simulink model "EV6_LUT_FourWheel_EV6Battery77p4kWh_PowerCorrected"  (R2024a)
settings: Solver=ode4  StartTime=0  StopTime=60  FixedStep=0.001  RelTol=1e-3
PreLoadFcn:
  | VSS_BICYCLE=Simulink.Variant('Dual=0');
  | VSS_DUAL=Simulink.Variant('Dual=1');
  | Dual=1;
  | load('DriveCycle2.mat')
PostLoadFcn:
  | if any(exist('dsrtsu_mdlpostloadfcn', 'file') ~= 0), dsrtsu_mdlpostloadfcn('Execute', bdroot); end
InitFcn:
  | , if any(exist('rtifpga_mdlclblib', 'file') ~= 0), rtifpga_mdlclblib('Init', bdroot); end,
  | , if any(exist('dsmpb_private', 'file') ~= 0), dsmpb_private('dsmpb_mdlclblib', 'Init', bdroot); end,
  | load('DriveCycle2.mat')
model workspace (MAT data in the model file):
  DiffRatio = 10.65
  EV6_2023_BattBranchCapacity_Ah = 55.5236728838
  EV6_2023_BattEnergy_kWh = 77.4
  EV6_2023_BattNominalVoltage_V = 697
  EV6_2023_BattNumCellsParallel = 2
  EV6_2023_BattNumCellsSeries = 192
  EV6_2023_BattOpenVoltCapBpts = [0 0.1 0.2 0.3 0.4 0.5 0.6 0.7 0.8 0.9 1]
  EV6_2023_BattOpenVoltTbl = [2.96762142548 3.40364281191 3.47417488548 3.54470541822 3.61523441014 3.68576186124 3.75628777151 3.82681214095 3.94527005036 4.07101207308 4.2120755254]
  EV6_2023_BattPackCapacity_Ah = 111.047345768
  EV6_2023_BattResistSocBpts = [0 0.2 0.4 0.6 0.8 1]
  EV6_2023_BattResistTbl = [0.0163620057716 0.0118174152018 0.00807187352333 0.00375663957972 0.00266904525531 0.00103635901355 0.0019014404175 0.0172368903217 0.0121226074867 0.00758541551769 0.00474065349228 0.00337561163613 ... (42 elements, 7x6)]
  EV6_2023_BattResistTempBpts = [243.1 253.1 263.1 273.1 283.1 298.1 313.1]
  EV6_2023_InitialPackOCV_V = 726.471714233
  EV6_2023_InitialSOC = 0.638878863672
  EV6_BattCellCapacity_Ah = 60.3
  EV6_BattInitialSOC = 0.638878863672
  EV6_BattOCV_Cell_V = [2.96762142548 3.40364281191 3.47417488548 3.54470541822 3.61523441014 3.68576186124 3.75628777151 3.82681214095 3.94527005036 4.07101207308 4.2120755254]
  EV6_BattOCV_SOC = [0 0.1 0.2 0.3 0.4 0.5 0.6 0.7 0.8 0.9 1]
  EV6_BattPackCapacity_Ah = 120.6
  EV6_BattParallelCells = 2
  EV6_BattResistanceSOC = [0 0.2 0.4 0.6 0.8 1]
  EV6_BattResistanceTable_Ohm = [0.0163620057716 0.0118174152018 0.00807187352333 0.00375663957972 0.00266904525531 0.00103635901355 0.0019014404175 0.0172368903217 0.0121226074867 0.00758541551769 0.00474065349228 0.00337561163613 ... (42 elements, 7x6)]
  EV6_BattResistanceTemp_K = [243.1 253.1 263.1 273.1 283.1 298.1 313.1]
  EV6_BattSeriesCells = 192
  EV6_FinalDriveRatio = 10.65
  EV6_TargetPackResistance_Ohm = 0.132763804608
  Gas = 0.383333333333
undefined symbols (not defined in the file): accel_bp_mps2, AccelCmd, ActTqLF_Nm_, ActTqLR_Nm_, ActTqRF_Nm_, ActTqRR_Nm_, BattChargeLimitMaxPwr, BattChargeLimitSocBpts, BattChargeLimitTbl, BattDischargeLimitSocBpts, BattDischargeLimitTbl, BattDischargeMaxPwr, BrakeMaxPrs, BrakeMaxTrq, ChassisDistCg2FrontAxle, ChassisDistCg2RearAxle, ChassisVehMass, CltchCmd, CoastDown, DecelCmd, DiscIntNeverNeededParam, EnvGravCnst, EnvPrs, EnvTemp, EV6_RegenTorqueGain, EV6_TractionTorqueGain, front_share_regen_3d, front_share_traction_3d, FuelSpecificGrav, GearCmd, h, InitStates, lgSw, limitedMCT, MCT, MtrEffSpdBpts, MtrEffTbl, MtrEffTrqBpts, MtrPwrMax, MtrTrqMax, out_1, pMCT, RealSimPara, Ref_speed, Ref_time, regen_torque_bp_Nm, speed_bp_kph, SteeringCmd, SupvsryCtrlRegenBrkCutOffTbl, SupvsryCtrlRegenSpdBpts, TestScnrioCycleNum, traction_torque_bp_Nm, US06, VEH
libraries: VSIGenLib x65, simulink x54, etargetslib x38, dsmpblib x24, vehdynlibtire x12, autolibshared x11, vehdynlibsuspension x7, vehdynlibtirecommon x7, autolibpowerinfoutils x6, autolibutils x5, autolibsharedcoupling x4, autolibmappedmotor x4
(part 10 of 19)

== system EV6_LUT_FourWheel_EV6Battery77p4kWh_PowerCorrected/Vehicle Under Test1/Vehicle/Powertrain Supervisory Controller /Engine Torque Command/Motor Torque Arbitration and Power Management/Power Management ==
  note: Power Management algorithm:
      | - Estimate Elec power based on mech power using efficiency map
      | - Check if Elec power is within battery power limits
      | - If power within limit , use motor torque command
      | - If power limit exceeded, use limited motor torque
      | - For low Mot Spd, MotPwrReq will be a small number.  Pass through torque command until Mot Spd > 2.
  BattPwrDischrgLmt : Inport
  BattPwrChrgLmt : Inport  Port=2
  MotSpd : Inport  Port=3
  MotTrqCmd : Inport  Port=4
  Abs : Abs  SaturateOnIntegerOverflow=off
  Check Within Limits : Subsystem
  Compare To Constant : simulink/Logic and Bit Operations/Compare To Constant  relop=<  const=2  OutDataTypeStr=boolean
  ElecToMechPwr : Product  Inputs=*/
  Mech to Elec Power Estimate : Subsystem
  MechPwrToTrq : Product  Inputs=*/
  Switch : Switch  Criteria=u2 > Threshold  SaturateOnIntegerOverflow=off  InputSameDT=off
  Switch1 : Switch  Criteria=u2 > Threshold  SaturateOnIntegerOverflow=off  InputSameDT=off
  Torque Limit : Subsystem
  div0protect - poly : autolibutils/div0protect - poly  thresh=2  ZeroCross1=on  aMode=aMode
  MotTrqCmdFinal : Outport  VectorParamsAs1DForOutWhenUnconnected=off
  wires:
  MotSpd/1 -> Torque Limit/2(MotSpd), div0protect - poly/1, Mech to Elec Power Estimate/2(MotSpd), Abs/1
  MotTrqCmd/1 -> Switch/1, Switch1/1, Mech to Elec Power Estimate/1(MotTrqCmd)
  div0protect - poly/1 -> MechPwrToTrq/2
  Mech to Elec Power Estimate/2(Eff2k) -> ElecToMechPwr/2
  ElecToMechPwr/1 -> MechPwrToTrq/1
  MechPwrToTrq/1 -> Switch/3
  Torque Limit/1(MotTrqCmd) -> MotTrqCmdFinal/1
  BattPwrDischrgLmt/1 -> Check Within Limits/1(up)
  Mech to Elec Power Estimate/1(MotPwrElecReq) -> Check Within Limits/2(u)
  BattPwrChrgLmt/1 -> Check Within Limits/3(lo)
  Check Within Limits/2(y) -> ElecToMechPwr/1
  Switch/1 -> Switch1/3
  Check Within Limits/1(InLimit) -> Switch/2
  Switch1/1 -> Torque Limit/1(MotTrq)
  Abs/1 -> Compare To Constant/1
  Compare To Constant/1 -> Switch1/2

== system EV6_LUT_FourWheel_EV6Battery77p4kWh_PowerCorrected/Vehicle Under Test1/Vehicle/Rototest and ORNL Interface/From Rototest/RotoTestEthRX/Depacker ==
  SysStsBits : Inport
  Extract Bits1 : simulink/Logic and Bit Operations/Extract Bits  bitsToExtract=Range of bits  numBits=8  bitIdxRange=[7]  outScalingMode=Preserve fixed-point scaling
  Extract Bits10 : simulink/Logic and Bit Operations/Extract Bits  bitsToExtract=Range of bits  numBits=8  bitIdxRange=[9]  outScalingMode=Preserve fixed-point scaling
  Extract Bits11 : simulink/Logic and Bit Operations/Extract Bits  bitsToExtract=Range of bits  numBits=8  bitIdxRange=[10]  outScalingMode=Preserve fixed-point scaling
  Extract Bits12 : simulink/Logic and Bit Operations/Extract Bits  bitsToExtract=Range of bits  numBits=8  bitIdxRange=[11]  outScalingMode=Preserve fixed-point scaling
  Extract Bits13 : simulink/Logic and Bit Operations/Extract Bits  bitsToExtract=Range of bits  numBits=8  bitIdxRange=[12]  outScalingMode=Preserve fixed-point scaling
  Extract Bits14 : simulink/Logic and Bit Operations/Extract Bits  bitsToExtract=Range of bits  numBits=8  bitIdxRange=[13]  outScalingMode=Preserve fixed-point scaling
  Extract Bits15 : simulink/Logic and Bit Operations/Extract Bits  bitsToExtract=Range of bits  numBits=8  bitIdxRange=[14]  outScalingMode=Preserve fixed-point scaling
  Extract Bits16 : simulink/Logic and Bit Operations/Extract Bits  bitsToExtract=Range of bits  numBits=8  bitIdxRange=[15]  outScalingMode=Preserve fixed-point scaling
  Extract Bits2 : simulink/Logic and Bit Operations/Extract Bits  bitsToExtract=Range of bits  numBits=8  bitIdxRange=[6]  outScalingMode=Preserve fixed-point scaling
  Extract Bits3 : simulink/Logic and Bit Operations/Extract Bits  bitsToExtract=Range of bits  numBits=8  bitIdxRange=[5]  outScalingMode=Preserve fixed-point scaling
  Extract Bits4 : simulink/Logic and Bit Operations/Extract Bits  bitsToExtract=Range of bits  numBits=8  bitIdxRange=[4]  outScalingMode=Preserve fixed-point scaling
  Extract Bits5 : simulink/Logic and Bit Operations/Extract Bits  bitsToExtract=Range of bits  numBits=8  bitIdxRange=[3]  outScalingMode=Preserve fixed-point scaling
  Extract Bits6 : simulink/Logic and Bit Operations/Extract Bits  bitsToExtract=Range of bits  numBits=8  bitIdxRange=[2]  outScalingMode=Preserve fixed-point scaling
  Extract Bits7 : simulink/Logic and Bit Operations/Extract Bits  bitsToExtract=Range of bits  numBits=8  bitIdxRange=[1]  outScalingMode=Preserve fixed-point scaling
  Extract Bits8 : simulink/Logic and Bit Operations/Extract Bits  bitsToExtract=Range of bits  numBits=8  bitIdxRange=[0]  outScalingMode=Preserve fixed-point scaling
  Extract Bits9 : simulink/Logic and Bit Operations/Extract Bits  bitsToExtract=Range of bits  numBits=8  bitIdxRange=[8]  outScalingMode=Preserve fixed-point scaling
  Gain : Gain  Gain=1/128
  Gain1 : Gain  Gain=1/64
  Gain10 : Gain  Gain=1/1024
  Gain11 : Gain  Gain=1/2048
  Gain12 : Gain  Gain=1/4096
  Gain13 : Gain  Gain=1/8192
  Gain14 : Gain  Gain=1/16384
  Gain15 : Gain  Gain=1/32768
  Gain2 : Gain  Gain=1/32
  Gain3 : Gain  Gain=1/16
  Gain4 : Gain  Gain=1/8
  Gain5 : Gain  Gain=1/4
  Gain6 : Gain  Gain=1/2
  Gain7 : Gain  Gain=1/1
  Gain8 : Gain  Gain=1/256
  Gain9 : Gain  Gain=1/512
  Header : VSIGenLib/Header  not=''
  Terminator{,1..8} (9 alike) : Terminator
  FaultActive : Outport
  WarningsActive : Outport  Port=2
  SpTqRR : Outport  Port=3
  SpTqLR : Outport  Port=4
  SpTqRF : Outport  Port=5
  SpTqLF : Outport  Port=6
  SystemActive : Outport  Port=7
  wires:
  Extract Bits6/1 -> Gain5/1
  Extract Bits4/1 -> Gain3/1
  Extract Bits8/1 -> Gain7/1
  Extract Bits7/1 -> Gain6/1
  Extract Bits3/1 -> Gain2/1
  Extract Bits1/1 -> Gain/1
  Extract Bits5/1 -> Gain4/1
  Extract Bits2/1 -> Gain1/1
  Extract Bits10/1 -> Gain9/1
  Extract Bits9/1 -> Gain8/1
  Extract Bits11/1 -> Gain10/1
  Extract Bits12/1 -> Gain11/1
  Extract Bits13/1 -> Gain12/1
  Extract Bits15/1 -> Gain14/1
  Extract Bits14/1 -> Gain13/1
  Extract Bits16/1 -> Gain15/1
  SysStsBits/1 -> Extract Bits1/1, Extract Bits2/1, Extract Bits3/1, Extract Bits4/1, Extract Bits5/1, Extract Bits6/1, Extract Bits7/1, Extract Bits8/1, Extract Bits11/1, Extract Bits12/1, Extract Bits13/1, Extract Bits14/1, Extract Bits15/1, Extract Bits16/1, Extract Bits10/1, Extract Bits9/1
  Gain15/1 -> Terminator6/1  "Reserved"
  Gain13/1 -> Terminator8/1  "Reserved"
  Gain14/1 -> Terminator7/1  "Reserved"
  Gain12/1 -> SpTqRR/1  "SpTqRR"
  Gain11/1 -> SpTqLR/1  "SpTqLR"
  Gain10/1 -> SpTqRF/1  "SpTqRF"
  Gain9/1 -> SpTqLF/1  "SpTqLF"
  Gain8/1 -> SystemActive/1  "SystemActive"
  Gain7/1 -> Terminator5/1  "Reserved"
  Gain/1 -> FaultActive/1  "FaultActive"
  Gain1/1 -> WarningsActive/1  "WarningsActive"
  Gain2/1 -> Terminator/1  "Reserved"
  Gain4/1 -> Terminator2/1  "Reserved"
  Gain3/1 -> Terminator1/1  "Reserved"
  Gain6/1 -> Terminator4/1  "Reserved"
  Gain5/1 -> Terminator3/1  "Reserved"

== system EV6_LUT_FourWheel_EV6Battery77p4kWh_PowerCorrected/Vehicle Under Test1/Vehicle/Rototest and ORNL Interface/Get Wheel Spd Cmd Based on Wheel Dynamics/Whl Dynamics & Format CM Powertrain Signal/Diff Trq ==
  In1 : Inport
  Constant : Constant  Value=4.1
  Gain10 : Gain  Gain=0.5
  Product : Product  RndMeth=Zero
  Out1 : Outport
  wires:
  Product/1 -> Gain10/1  "DiffTrq"
  In1/1 -> Product/2
  Constant/1 -> Product/1
  Gain10/1 -> Out1/1

== system EV6_LUT_FourWheel_EV6Battery77p4kWh_PowerCorrected/Vehicle Under Test1/Vehicle/Rototest and ORNL Interface/Get Wheel Spd Cmd Based on Wheel Dynamics/Whl Dynamics & Format CM Powertrain Signal/Subsystem ==
  BrakeTorq : Inport
  <Car Trq_T2WFL> : Inport  Port=2
  AxlTorq : Inport  Port=3
  Fx : Inport  Port=4
  Add1 : Sum  Inputs=--+
  Add2 : Sum  Inputs=-+
  Constant : Constant  Value=0
  Constant9 : Constant  Value=0.3135
  MATLAB Function : MATLAB Function  TreatAsAtomicUnit=on
  Memory : Memory
  Output Damping : Gain  Gain=0  SaturateOnIntegerOverflow=on  OutDataTypeStr=Inherit: Same as input  ParamDataTypeStr=Inherit: Same as input
  Product3 : Product  Inputs=**
  Saturation : Saturate  UpperLimit=inf  LowerLimit=0  ZeroCross=off
  Sum : Sum  Inputs=--
  Sum3 : Sum  Inputs=-++
  Switch : Switch  Criteria=u2 > Threshold  SaturateOnIntegerOverflow=off  InputSameDT=off
  WheelInertia : Subsystem
  WheelInertia1 : Subsystem
  omega wheel : Integrator  ContinuousStateAttributes='omegaWheel'
  rotv FL : Outport
  wires:
  [Fx1] -> Product3/1
  Sum/1 -> Switch/3
  WheelInertia1/1(axleTorq) -> Sum/1  "rota"
  Output Damping/1 -> Sum/2
  omega wheel/1 -> rotv FL/1, Output Damping/1, Memory/1
  Switch/1 -> omega wheel/1
  Add1/1 -> WheelInertia1/1(In1)
  Saturation/1 -> Product3/2
  Product3/1 -> Add1/3
  <Car Trq_T2WFL>/1 -> Sum3/2, Add1/2
  AxlTorq/1 -> Sum3/3, MATLAB Function/1(axleTorq), Add1/1
  Constant9/1 -> Add2/2
  [RhoZ1] -> Add2/1
  Add2/1 -> Saturation/1
  Memory/1 -> MATLAB Function/2(wheelSpd)
  Constant/1 -> Switch/1
  MATLAB Function/1(switchFlag) -> Switch/2  "Flag1"
  BrakeTorq/1 -> Sum3/1
  Sum3/1 -> WheelInertia/1(In1)

== system EV6_LUT_FourWheel_EV6Battery77p4kWh_PowerCorrected/Vehicle Under Test1/Vehicle/Rototest and ORNL Interface/Get Wheel Spd Cmd Based on Wheel Dynamics/Whl Dynamics & Format CM Powertrain Signal/Subsystem1 ==
  BrakeTorq : Inport
  <Car Trq_T2WFL> : Inport  Port=2
  AxlTorq : Inport  Port=3
  Discrete-Time Integrator : DiscreteIntegrator  IntegratorMethod=Integration: Backward Euler  InitialCondition=0/3.6/0.3235  SampleTime=0.001  ICPrevOutput=DiscIntNeverNeededParam  ICPrevScaledInput=DiscIntNeverNeededParam
  Sum3 : Sum  Inputs=-++
  WheelInertia : Subsystem
  rotv FL : Outport
  wires:
  WheelInertia/1(Out1) -> Discrete-Time Integrator/1
  Discrete-Time Integrator/1 -> rotv FL/1  "rotv FL"
  BrakeTorq/1 -> Sum3/1
  <Car Trq_T2WFL>/1 -> Sum3/2
  AxlTorq/1 -> Sum3/3
  Sum3/1 -> WheelInertia/1(In1)

== system EV6_LUT_FourWheel_EV6Battery77p4kWh_PowerCorrected/Vehicle Under Test1/Vehicle/Rototest and ORNL Interface/Get Wheel Spd Cmd Based on Wheel Dynamics/Whl Dynamics & Format CM Powertrain Signal/Subsystem2 ==
  BrakeTorq : Inport
  <Car Trq_T2WFR> : Inport  Port=2
  AxlTorq : Inport  Port=3
  Fx : Inport  Port=4
  Add1 : Sum  Inputs=--+
  Add2 : Sum  Inputs=-+
  Constant : Constant  Value=0
  Constant9 : Constant  Value=0.3135
  MATLAB Function : MATLAB Function  TreatAsAtomicUnit=on
  Memory : Memory
  Output Damping : Gain  Gain=-1  SaturateOnIntegerOverflow=on  OutDataTypeStr=Inherit: Same as input  ParamDataTypeStr=Inherit: Same as input
  Product3 : Product  Inputs=**
  Saturation : Saturate  UpperLimit=inf  LowerLimit=0  ZeroCross=off
  Sum3 : Sum  Inputs=-++
  Switch : Switch  Criteria=u2 > Threshold  SaturateOnIntegerOverflow=off  InputSameDT=off
  WheelInertia : Subsystem
  WheelInertia1 : Subsystem
  omega wheel : Integrator  ContinuousStateAttributes='omegaWheel'
  rotv FR : Outport
  wires:
  [Fx2] -> Product3/1
  Output Damping/1 -> Switch/3
  Switch/1 -> omega wheel/1
  omega wheel/1 -> rotv FR/1, Memory/1
  AxlTorq/1 -> Sum3/3, MATLAB Function/1(axleTorq), Add1/1
  Add2/1 -> Saturation/1
  Saturation/1 -> Product3/2
  [RhoZ2] -> Add2/1
  Add1/1 -> WheelInertia1/1(In1)
  Constant9/1 -> Add2/2
  <Car Trq_T2WFR>/1 -> Sum3/2, Add1/2
  Product3/1 -> Add1/3
  WheelInertia1/1(Out1) -> Output Damping/1  "rota"
  Memory/1 -> MATLAB Function/2(wheelSpd)
  Sum3/1 -> WheelInertia/1(In1)
  BrakeTorq/1 -> Sum3/1
  Constant/1 -> Switch/1
  MATLAB Function/1(switchFlag) -> Switch/2

== system EV6_LUT_FourWheel_EV6Battery77p4kWh_PowerCorrected/Vehicle Under Test1/Vehicle/Rototest and ORNL Interface/Get Wheel Spd Cmd Based on Wheel Dynamics/Whl Dynamics & Format CM Powertrain Signal/Subsystem3 ==
  BrakeTorq : Inport
  <Car Trq_T2WRL> : Inport  Port=2
  AxlTorq : Inport  Port=3
  Fx : Inport  Port=4
  FWSpd : Inport  Port=5
  Add1 : Sum  Inputs=--+
  Add2 : Sum  Inputs=-+
  Constant : Constant  Value=0
  Constant9 : Constant  Value=0.3135
  MATLAB Function : MATLAB Function  TreatAsAtomicUnit=on
  Memory : Memory
  Output Damping : Gain  Gain=0  SaturateOnIntegerOverflow=on  OutDataTypeStr=Inherit: Same as input  ParamDataTypeStr=Inherit: Same as input
  Product3 : Product  Inputs=**
  Saturation : Saturate  UpperLimit=inf  LowerLimit=0  ZeroCross=off
  Sum : Sum  Inputs=--
  Sum3 : Sum  Inputs=-++
  Switch : Switch  Criteria=u2 > Threshold  SaturateOnIntegerOverflow=off  InputSameDT=off
  WheelInertia : Subsystem
  WheelInertia1 : Subsystem
  omega wheel : Integrator  ContinuousStateAttributes='omegaWheel'
  rotv RL : Outport
  wires:
  WheelInertia1/1(axleTorq) -> Sum/1  "rota"
  omega wheel/1 -> rotv RL/1, Output Damping/1
  Output Damping/1 -> Sum/2
  [Fx3] -> Product3/1
  Switch/1 -> omega wheel/1
  Sum/1 -> Switch/3
  FWSpd/1 -> MATLAB Function/2(wheelSpd)
  AxlTorq/1 -> Sum3/3, MATLAB Function/1(axleTorq), Add1/1
  Add2/1 -> Saturation/1
  Saturation/1 -> Product3/2
  [RhoZ3] -> Add2/1
  Add1/1 -> WheelInertia1/1(In1)
  Constant9/1 -> Add2/2
  <Car Trq_T2WRL>/1 -> Add1/2, Sum3/2
  Product3/1 -> Add1/3
  Sum3/1 -> WheelInertia/1(In1)
  BrakeTorq/1 -> Sum3/1
  Constant/1 -> Switch/1
  MATLAB Function/1(switchFlag) -> Switch/2

== system EV6_LUT_FourWheel_EV6Battery77p4kWh_PowerCorrected/Vehicle Under Test1/Vehicle/Rototest and ORNL Interface/Get Wheel Spd Cmd Based on Wheel Dynamics/Whl Dynamics & Format CM Powertrain Signal/Subsystem4 ==
  BrakeTorq : Inport
  <Car Trq_T2WRR> : Inport  Port=2
  AxlTorq : Inport  Port=3
  Fx : Inport  Port=4
  FWSpd : Inport  Port=5
  Add1 : Sum  Inputs=--+
  Add2 : Sum  Inputs=-+
  Constant : Constant  Value=0
  Constant9 : Constant  Value=0.3135
  Gain : Gain  Gain=-1
  MATLAB Function : MATLAB Function  TreatAsAtomicUnit=on
  Memory : Memory
  Product3 : Product  Inputs=**
  Saturation : Saturate  UpperLimit=inf  LowerLimit=0  ZeroCross=off
  Sum3 : Sum  Inputs=-++
  Switch : Switch  Criteria=u2 > Threshold  SaturateOnIntegerOverflow=off  InputSameDT=off
  WheelInertia : Subsystem
  WheelInertia1 : Subsystem
  omega wheel : Integrator  ContinuousStateAttributes='omegaWheel'
  rotv RR : Outport
  wires:
  WheelInertia1/1(axleTorq) -> Gain/1  "rota"
  [Fx4] -> Product3/1
  omega wheel/1 -> rotv RR/1
  Switch/1 -> omega wheel/1
  Gain/1 -> Switch/3
  FWSpd/1 -> MATLAB Function/2(wheelSpd)
  AxlTorq/1 -> Sum3/3, MATLAB Function/1(axleTorq), Add1/1
  Add2/1 -> Saturation/1
  Saturation/1 -> Product3/2
  [RhoZ4] -> Add2/1
  Add1/1 -> WheelInertia1/1(In1)
  Constant9/1 -> Add2/2
  <Car Trq_T2WRR>/1 -> Sum3/2, Add1/2
  Product3/1 -> Add1/3
  Sum3/1 -> WheelInertia/1(In1)
  BrakeTorq/1 -> Sum3/1
  Constant/1 -> Switch/1
  MATLAB Function/1(switchFlag) -> Switch/2

== system EV6_LUT_FourWheel_EV6Battery77p4kWh_PowerCorrected/Vehicle Under Test1/Vehicle/Rototest and ORNL Interface/Get Wheel Spd Cmd Based on Wheel Dynamics/Whl Dynamics & Format CM Powertrain Signal/Subsystem5 ==
  In1 : Inport
  <Car Trq_T2WFR> : Inport  Port=2
  In3 : Inport  Port=3
  Discrete-Time Integrator1 : DiscreteIntegrator  IntegratorMethod=Integration: Backward Euler  InitialCondition=0/3.6/0.3235  SampleTime=0.001  ICPrevOutput=DiscIntNeverNeededParam  ICPrevScaledInput=DiscIntNeverNeededParam
  Sum2 : Sum  Inputs=-++
  WheelInertia1 : Subsystem
  rotv FR : Outport
  wires:
  Discrete-Time Integrator1/1 -> rotv FR/1  "rotv FR"
  In1/1 -> Sum2/1
  WheelInertia1/1(Out1) -> Discrete-Time Integrator1/1  "rota"
  In3/1 -> Sum2/3
  Sum2/1 -> WheelInertia1/1(In1)
  <Car Trq_T2WFR>/1 -> Sum2/2

== system EV6_LUT_FourWheel_EV6Battery77p4kWh_PowerCorrected/Vehicle Under Test1/Vehicle/Rototest and ORNL Interface/Get Wheel Spd Cmd Based on Wheel Dynamics/Whl Dynamics & Format CM Powertrain Signal/Subsystem6 ==
  In1 : Inport
  <Car Trq_T2WRL> : Inport  Port=2
  In3 : Inport  Port=3
  Discrete-Time Integrator2 : DiscreteIntegrator  IntegratorMethod=Integration: Backward Euler  InitialCondition=0/3.6/0.3235  SampleTime=0.001  ICPrevOutput=DiscIntNeverNeededParam  ICPrevScaledInput=DiscIntNeverNeededParam
  Sum : Sum  Inputs=-++
  WheelInertia2 : Subsystem
  rotv RL : Outport
  wires:
  In1/1 -> Sum/1
  Discrete-Time Integrator2/1 -> rotv RL/1  "rotv RL"
  Sum/1 -> WheelInertia2/1(In1)
  <Car Trq_T2WRL>/1 -> Sum/2
  WheelInertia2/1(Out1) -> Discrete-Time Integrator2/1  "rota"
  In3/1 -> Sum/3

== system EV6_LUT_FourWheel_EV6Battery77p4kWh_PowerCorrected/Vehicle Under Test1/Vehicle/Rototest and ORNL Interface/Get Wheel Spd Cmd Based on Wheel Dynamics/Whl Dynamics & Format CM Powertrain Signal/Subsystem7 ==
  In1 : Inport
  <Car Trq_T2WRR> : Inport  Port=2
  In3 : Inport  Port=3
  Discrete-Time Integrator3 : DiscreteIntegrator  IntegratorMethod=Integration: Backward Euler  InitialCondition=0/3.6/0.3235  SampleTime=0.001  ICPrevOutput=DiscIntNeverNeededParam  ICPrevScaledInput=DiscIntNeverNeededParam
  Sum1 : Sum  Inputs=-++
  WheelInertia3 : Subsystem
  rotv RR : Outport
  wires:
  Discrete-Time Integrator3/1 -> rotv RR/1  "rotv RR"
  In1/1 -> Sum1/1
  <Car Trq_T2WRR>/1 -> Sum1/2
  In3/1 -> Sum1/3
  WheelInertia3/1(Out1) -> Discrete-Time Integrator3/1  "rota"
  Sum1/1 -> WheelInertia3/1(In1)

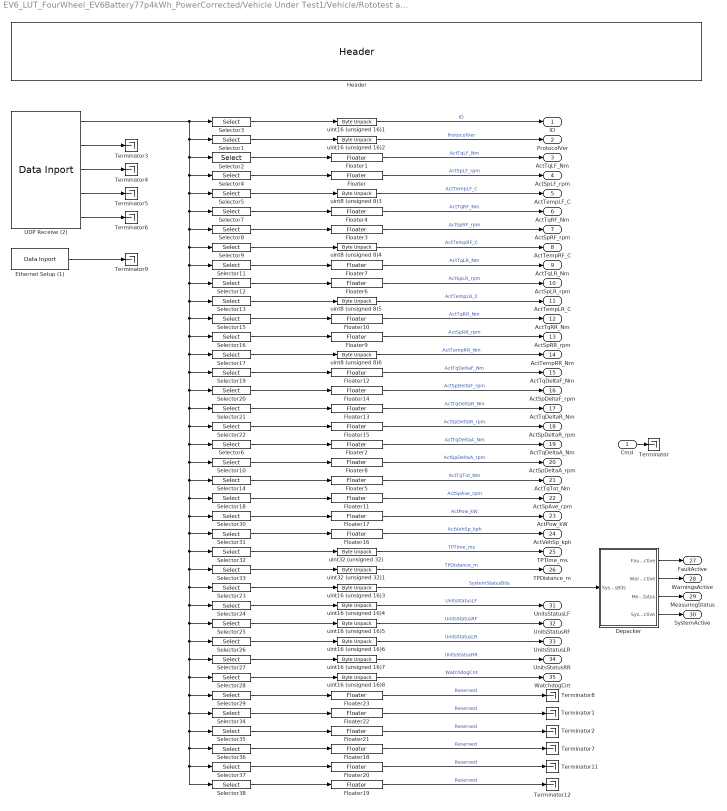
== system EV6_LUT_FourWheel_EV6Battery77p4kWh_PowerCorrected/Vehicle Under Test1/Vehicle/Rototest and ORNL Interface/To Rototest with Band-Aid/Logging/RotoTestEthRXLogging ==
  Cmd : Inport
  Depacker : Subsystem
  Ethernet Setup (1) : dsmpblib/Data Inport  Priority=10000
      settings: SourceProductName=dSPACE Model Interface Package for Simulink (MIPS)
  Floater{,1..23} (24 alike) : VSIGenLib/Floater  SystemSampleTime=-1  VariantActivationTime=update diagram  AllowFlexibleInterface=on  Latency=0  AutoFrameSizeCalculation=off
  Header : VSIGenLib/Header  not=''
  Selector1 : Selector  IndexMode=Zero-based  InputPortWidth=124  IndexOptions=Index vector (dialog)  Indices=[3 2]  OutputSizes=1
  Selector10 : Selector  IndexMode=Zero-based  InputPortWidth=124  IndexOptions=Index vector (dialog)  Indices=[63 62 61 60]  OutputSizes=1
  Selector11 : Selector  IndexMode=Zero-based  InputPortWidth=124  IndexOptions=Index vector (dialog)  Indices=[25 24 23 22]  OutputSizes=1
  Selector12 : Selector  IndexMode=Zero-based  InputPortWidth=124  IndexOptions=Index vector (dialog)  Indices=[29 28 27 26]  OutputSizes=1
  Selector13 : Selector  IndexMode=Zero-based  InputPortWidth=124  IndexOptions=Index vector (dialog)  Indices=[30]  OutputSizes=1
  Selector14 : Selector  IndexMode=Zero-based  InputPortWidth=124  IndexOptions=Index vector (dialog)  Indices=[67 66 65 64]  OutputSizes=1
  Selector15 : Selector  IndexMode=Zero-based  InputPortWidth=124  IndexOptions=Index vector (dialog)  Indices=[34 33 32 31]  OutputSizes=1
  Selector16 : Selector  IndexMode=Zero-based  InputPortWidth=124  IndexOptions=Index vector (dialog)  Indices=[38 37 36 35]  OutputSizes=1
  Selector17 : Selector  IndexMode=Zero-based  InputPortWidth=124  IndexOptions=Index vector (dialog)  Indices=[39]  OutputSizes=1
  Selector18 : Selector  IndexMode=Zero-based  InputPortWidth=124  IndexOptions=Index vector (dialog)  Indices=[71 70 69 68]  OutputSizes=1
  Selector19 : Selector  IndexMode=Zero-based  InputPortWidth=124  IndexOptions=Index vector (dialog)  Indices=[43 42 41 40]  OutputSizes=1
  Selector2 : Selector  IndexMode=Zero-based  InputPortWidth=124  IndexOptions=Index vector (dialog)  Indices=[7 6 5 4]  OutputSizes=1
  Selector20 : Selector  IndexMode=Zero-based  InputPortWidth=124  IndexOptions=Index vector (dialog)  Indices=[47 46 45 44]  OutputSizes=1
  Selector21 : Selector  IndexMode=Zero-based  InputPortWidth=124  IndexOptions=Index vector (dialog)  Indices=[51 50 49 48]  OutputSizes=1
  Selector22 : Selector  IndexMode=Zero-based  InputPortWidth=124  IndexOptions=Index vector (dialog)  Indices=[55 54 53 52]  OutputSizes=1
  Selector23 : Selector  IndexMode=Zero-based  InputPortWidth=124  IndexOptions=Index vector (dialog)  Indices=[89 88]  OutputSizes=1
  Selector24 : Selector  IndexMode=Zero-based  InputPortWidth=124  IndexOptions=Index vector (dialog)  Indices=[91 90]  OutputSizes=1
  Selector25 : Selector  IndexMode=Zero-based  InputPortWidth=124  IndexOptions=Index vector (dialog)  Indices=[93 92]  OutputSizes=1
  Selector26 : Selector  IndexMode=Zero-based  InputPortWidth=124  IndexOptions=Index vector (dialog)  Indices=[95 94]  OutputSizes=1
  Selector27 : Selector  IndexMode=Zero-based  InputPortWidth=124  IndexOptions=Index vector (dialog)  Indices=[97 96]  OutputSizes=1
  Selector28 : Selector  IndexMode=Zero-based  InputPortWidth=124  IndexOptions=Index vector (dialog)  Indices=[99 98]  OutputSizes=1
  Selector29 : Selector  IndexMode=Zero-based  InputPortWidth=124  IndexOptions=Index vector (dialog)  Indices=[103 102 101 100]  OutputSizes=1
  Selector3 : Selector  IndexMode=Zero-based  InputPortWidth=124  IndexOptions=Index vector (dialog)  Indices=[1 0]  OutputSizes=1
  Selector30 : Selector  IndexMode=Zero-based  InputPortWidth=124  IndexOptions=Index vector (dialog)  Indices=[67 66 65 64]  OutputSizes=1
  Selector31 : Selector  IndexMode=Zero-based  InputPortWidth=124  IndexOptions=Index vector (dialog)  Indices=[71 70 69 68]  OutputSizes=1
  Selector32 : Selector  IndexMode=Zero-based  InputPortWidth=124  IndexOptions=Index vector (dialog)  Indices=[83 82 81 80]  OutputSizes=1
  Selector33 : Selector  IndexMode=Zero-based  InputPortWidth=124  IndexOptions=Index vector (dialog)  Indices=[87 86 85 84]  OutputSizes=1
  Selector34 : Selector  IndexMode=Zero-based  InputPortWidth=124  IndexOptions=Index vector (dialog)  Indices=[107 106 105 104]  OutputSizes=1
  Selector35 : Selector  IndexMode=Zero-based  InputPortWidth=124  IndexOptions=Index vector (dialog)  Indices=[111 110 109 108]  OutputSizes=1
  Selector36 : Selector  IndexMode=Zero-based  InputPortWidth=124  IndexOptions=Index vector (dialog)  Indices=[115 114 113 112]  OutputSizes=1
  Selector37 : Selector  IndexMode=Zero-based  InputPortWidth=124  IndexOptions=Index vector (dialog)  Indices=[119 118 117 116]  OutputSizes=1
  Selector38 : Selector  IndexMode=Zero-based  InputPortWidth=124  IndexOptions=Index vector (dialog)  Indices=[123 122 121 120]  OutputSizes=1
  Selector4 : Selector  IndexMode=Zero-based  InputPortWidth=124  IndexOptions=Index vector (dialog)  Indices=[11 10 9 8]  OutputSizes=1
  Selector5 : Selector  IndexMode=Zero-based  InputPortWidth=124  IndexOptions=Index vector (dialog)  Indices=[12]  OutputSizes=1
  Selector6 : Selector  IndexMode=Zero-based  InputPortWidth=124  IndexOptions=Index vector (dialog)  Indices=[59 58 57 56]  OutputSizes=1
  Selector7 : Selector  IndexMode=Zero-based  InputPortWidth=124  IndexOptions=Index vector (dialog)  Indices=[16 15 14 13]  OutputSizes=1
  Selector8 : Selector  IndexMode=Zero-based  InputPortWidth=124  IndexOptions=Index vector (dialog)  Indices=[20 19 18 17]  OutputSizes=1
  Selector9 : Selector  IndexMode=Zero-based  InputPortWidth=124  IndexOptions=Index vector (dialog)  Indices=[21]  OutputSizes=1
  Terminator{,1..9,11..12} (12 alike) : Terminator
  UDP Receive (2) : dsmpblib/Data Inport  Priority=10000
      settings: SourceProductName=dSPACE Model Interface Package for Simulink (MIPS)
  uint16 (unsigned 16){1..8} (8 alike) : etargetslib/Byte Unpack  dimensions={[1]}  datatypes={'uint16'}  byteAlign=1
  uint32 (unsigned 32) : etargetslib/Byte Unpack  dimensions={[1]}  datatypes={'uint32'}  byteAlign=1
  uint32 (unsigned 32)1 : etargetslib/Byte Unpack  dimensions={[1]}  datatypes={'uint32'}  byteAlign=1
  uint8 (unsigned 8){3..6} (4 alike) : etargetslib/Byte Unpack  dimensions={[1]}  datatypes={'uint8'}  byteAlign=1
  ID : Outport
  ProtocolVer : Outport  Port=2
  ActTqLF_Nm : Outport  Port=3
  ActSpLF_rpm : Outport  Port=4
  ActTempLF_C : Outport  Port=5
  ActTqRF_Nm : Outport  Port=6
  ActSpRF_rpm : Outport  Port=7
  ActTempRF_C : Outport  Port=8
  ActTqLR_Nm : Outport  Port=9
  ActSpLR_rpm : Outport  Port=10
  ActTempLR_C : Outport  Port=11
  ActTqRR_Nm : Outport  Port=12
  ActSpRR_rpm : Outport  Port=13
  ActTempRR_Nm : Outport  Port=14
  ActTqDeltaF_Nm : Outport  Port=15
  ActSpDeltaF_rpm : Outport  Port=16
  ActTqDeltaR_Nm : Outport  Port=17
  ActSpDeltaR_rpm : Outport  Port=18
  ActTqDeltaA_Nm : Outport  Port=19
  ActSpDeltaA_rpm : Outport  Port=20
  ActTqTot_Nm : Outport  Port=21
  ActSpAve_rpm : Outport  Port=22
  ActPow_kW : Outport  Port=23
  ActVehSp_kph : Outport  Port=24
  TPTime_ms : Outport  Port=25
  TPDistance_m : Outport  Port=26
  FaultActive : Outport  Port=27
  WarningsActive : Outport  Port=28
  MeasuringStatus : Outport  Port=29
  SystemActive : Outport  Port=30
  UnitsStatusLF : Outport  Port=31
  UnitsStatusRF : Outport  Port=32
  UnitsStatusLR : Outport  Port=33
  UnitsStatusRR : Outport  Port=34
  WatchdogCnt : Outport  Port=35
  wires:
  Cmd/1 -> Terminator/1
  Floater23/1 -> Terminator8/1  "Reserved"
  Floater22/1 -> Terminator1/1  "Reserved"
  Floater21/1 -> Terminator2/1  "Reserved"
  Floater20/1 -> Terminator11/1  "Reserved"
  Floater19/1 -> Terminator12/1  "Reserved"
  Floater18/1 -> Terminator7/1  "Reserved"
  Selector38/1 -> Floater19/1
  UDP Receive (2)/1 -> Selector7/1, Selector8/1, Selector9/1, Selector11/1, Selector12/1, Selector13/1, Selector15/1, Selector16/1, Selector17/1, Selector19/1, Selector20/1, Selector21/1, Selector22/1, Selector6/1, Selector10/1, Selector14/1, Selector18/1, Selector30/1, Selector31/1, Selector32/1, Selector33/1, Selector23/1, Selector25/1, Selector26/1, Selector27/1, Selector29/1, Selector34/1, Selector35/1, Selector36/1, Selector37/1, Selector38/1, Selector28/1, Selector24/1, Selector5/1, Selector4/1, Selector2/1, Selector1/1, Selector3/1
  Selector37/1 -> Floater20/1
  Selector36/1 -> Floater18/1
  Selector35/1 -> Floater21/1
  Selector34/1 -> Floater22/1
  Selector32/1 -> uint32 (unsigned 32)/1
  Selector33/1 -> uint32 (unsigned 32)1/1
  uint32 (unsigned 32)1/1 -> TPDistance_m/1  "TPDistance_m"
  uint32 (unsigned 32)/1 -> TPTime_ms/1  "TPTime_ms"
  Floater16/1 -> ActVehSp_kph/1  "ActVehSp_kph"
  Selector31/1 -> Floater16/1
  Floater17/1 -> ActPow_kW/1  "ActPow_kW"
  Selector30/1 -> Floater17/1
  Selector6/1 -> Floater2/1
  Selector14/1 -> Floater5/1
  Selector10/1 -> Floater8/1
  Floater5/1 -> ActTqTot_Nm/1  "ActTqTot_Nm"
  Selector18/1 -> Floater11/1
  Floater2/1 -> ActTqDeltaA_Nm/1  "ActTqDeltaA_Nm"
  Floater8/1 -> ActSpDeltaA_rpm/1  "ActSpDeltaA_rpm"
  Floater11/1 -> ActSpAve_rpm/1  "ActSpAve_rpm"
  Ethernet Setup (1)/1 -> Terminator9/1
  Depacker/4(SystemActive) -> SystemActive/1
  Depacker/1(FaultActive) -> FaultActive/1
  Depacker/2(WarningsActive) -> WarningsActive/1
  Depacker/3(MeasuringStatus) -> MeasuringStatus/1
  uint8 (unsigned 8)4/1 -> ActTempRF_C/1  "ActTempRF_C"
  Floater/1 -> ActSpLF_rpm/1  "ActSpLF_rpm"
  uint16 (unsigned 16)1/1 -> ID/1  "ID"
  Floater15/1 -> ActSpDeltaR_rpm/1  "ActSpDeltaR_rpm"
  uint16 (unsigned 16)8/1 -> WatchdogCnt/1  "WatchdogCnt"
  Floater14/1 -> ActSpDeltaF_rpm/1  "ActSpDeltaF_rpm"
  uint16 (unsigned 16)5/1 -> UnitsStatusRF/1  "UnitsStatusRF"
  Floater9/1 -> ActSpRR_rpm/1  "ActSpRR_rpm"
  Floater1/1 -> ActTqLF_Nm/1  "ActTqLF_Nm"
  uint8 (unsigned 8)3/1 -> ActTempLF_C/1  "ActTempLF_C"
  Floater12/1 -> ActTqDeltaF_Nm/1  "ActTqDeltaF_Nm"
  Floater7/1 -> ActTqLR_Nm/1  "ActTqLR_Nm"
  uint16 (unsigned 16)2/1 -> ProtocolVer/1  "ProtocolVer"
  Selector24/1 -> uint16 (unsigned 16)4/1
  Selector7/1 -> Floater4/1
  Selector8/1 -> Floater3/1
  uint16 (unsigned 16)7/1 -> UnitsStatusRR/1  "UnitsStatusRR"
  Selector22/1 -> Floater15/1
  Selector12/1 -> Floater6/1
  Selector23/1 -> uint16 (unsigned 16)3/1
  uint16 (unsigned 16)6/1 -> UnitsStatusLR/1  "UnitsStatusLR"
  Selector17/1 -> uint8 (unsigned 8)6/1
  UDP Receive (2)/3 -> Terminator4/1
  uint16 (unsigned 16)4/1 -> UnitsStatusLF/1  "UnitsStatusLF"
  Selector27/1 -> uint16 (unsigned 16)7/1
  Floater13/1 -> ActTqDeltaR_Nm/1  "ActTqDeltaR_Nm"
  Selector2/1 -> Floater1/1
  Selector13/1 -> uint8 (unsigned 8)5/1
  Selector26/1 -> uint16 (unsigned 16)6/1
  uint16 (unsigned 16)3/1 -> Depacker/1(SysStsBits)  "SystemStatusBits"
  Floater3/1 -> ActSpRF_rpm/1  "ActSpRF_rpm"
  UDP Receive (2)/2 -> Terminator3/1
  Selector25/1 -> uint16 (unsigned 16)5/1
  Floater4/1 -> ActTqRF_Nm/1  "ActTqRF_Nm"
  Selector29/1 -> Floater23/1
  uint8 (unsigned 8)6/1 -> ActTempRR_Nm/1  "ActTempRR_Nm"
  Floater6/1 -> ActSpLR_rpm/1  "ActSpLR_rpm"
  Selector20/1 -> Floater14/1
  Selector9/1 -> uint8 (unsigned 8)4/1
  Selector5/1 -> uint8 (unsigned 8)3/1
  Selector15/1 -> Floater10/1
  Selector16/1 -> Floater9/1
  uint8 (unsigned 8)5/1 -> ActTempLR_C/1  "ActTempLR_C"
  Selector3/1 -> uint16 (unsigned 16)1/1
  UDP Receive (2)/4 -> Terminator5/1
  Selector28/1 -> uint16 (unsigned 16)8/1
  Selector21/1 -> Floater13/1
  Selector19/1 -> Floater12/1
  Selector1/1 -> uint16 (unsigned 16)2/1
  UDP Receive (2)/5 -> Terminator6/1
  Selector4/1 -> Floater/1
  Floater10/1 -> ActTqRR_Nm/1  "ActTqRR_Nm"
  Selector11/1 -> Floater7/1

== system EV6_LUT_FourWheel_EV6Battery77p4kWh_PowerCorrected/Vehicle Under Test1/Vehicle/Rototest and ORNL Interface/To Rototest with Band-Aid/RotoTestEthTx/Packer ==
  SpTqRR : Inport
  SpTqLR : Inport  Port=2
  SpTqRF : Inport  Port=3
  SpTqLF : Inport  Port=4
  SystemActive : Inport  Port=5
  Add : Sum  Inputs=++++++++  OutDataTypeStr=uint8
  Bit0 : Gain  OutDataTypeStr=uint8
  Bit1 : Gain  Gain=2  OutDataTypeStr=uint8
  Bit2 : Gain  Gain=4  OutDataTypeStr=Inherit: Inherit via back propagation
  Bit3 : Gain  Gain=8  OutDataTypeStr=uint8
  Bit4 : Gain  Gain=16  OutDataTypeStr=uint8
  Bit5 : Gain  Gain=32  OutDataTypeStr=uint8
  Bit6 : Gain  Gain=64  OutDataTypeStr=uint8
  Bit7 : Gain  Gain=128  OutDataTypeStr=uint8
  Ground11 : Ground
  Header : VSIGenLib/Header  not=''
  SystemCtrlBits : Outport
  wires:
  SpTqRF/1 -> Bit2/1
  SpTqLF/1 -> Bit1/1
  SpTqRR/1 -> Bit4/1
  SpTqLR/1 -> Bit3/1
  Add/1 -> SystemCtrlBits/1  "SystemCtrlBits"
  Bit0/1 -> Add/8  "SystemActive"
  Bit1/1 -> Add/7  "SpTqLF"
  Bit7/1 -> Add/1  "Reserved"
  SystemActive/1 -> Bit0/1
  Bit4/1 -> Add/4  "SpTqRR"
  Bit6/1 -> Add/2  "Reserved"
  Bit3/1 -> Add/5  "SpTqLR"
  Ground11/1 -> Bit7/1, Bit5/1, Bit6/1  "Reserved"
  Bit5/1 -> Add/3  "Reserved"
  Bit2/1 -> Add/6  "SpTqRF"

== system EV6_LUT_FourWheel_EV6Battery77p4kWh_PowerCorrected/Vehicle Under Test1/Vehicle/Vehicle Dynamics/Vehicle 14DOF/Subsystem1/Subsystem ==
  Cgxyzdot : Inport
  angles : Inport  Port=2
  Demux2 : Demux  Outputs=3
  Demux3 : Demux  Outputs=3
  Scope : Scope
  Terminator{,1..4} (5 alike) : Terminator
  VehSpd : Outport
  wires:
  Cgxyzdot/1 -> Demux2/1
  Demux3/2 -> Terminator3/1  "theta"
  Demux2/2 -> Scope/1, Terminator/1  "xdot"
  Demux3/1 -> Terminator2/1  "phi"
  Demux3/3 -> Terminator4/1  "psi"
  Demux2/3 -> Terminator1/1  "zdot"
  angles/1 -> Demux3/1
  Demux2/1 -> VehSpd/1  "xdot"

== system EV6_LUT_FourWheel_EV6Battery77p4kWh_PowerCorrected/Vehicle Under Test1/Vehicle/Vehicle Dynamics/Vehicle 14DOF/Subsystem4/Subsystem ==
  Cgxyzdot : Inport
  angles : Inport  Port=2
  Demux2 : Demux  Outputs=3
  Demux3 : Demux  Outputs=3
  Terminator{,1..4} (5 alike) : Terminator
  VehSpd : Outport
  wires:
  Demux2/1 -> VehSpd/1  "xdot"
  angles/1 -> Demux3/1
  Demux2/3 -> Terminator1/1  "zdot"
  Demux3/3 -> Terminator4/1  "psi"
  Demux3/1 -> Terminator2/1  "phi"
  Demux2/2 -> Terminator/1  "xdot"
  Demux3/2 -> Terminator3/1  "theta"
  Cgxyzdot/1 -> Demux2/1

== system EV6_LUT_FourWheel_EV6Battery77p4kWh_PowerCorrected/Vehicle Under Test1/Vehicle/Vehicle Dynamics/Vehicle 14DOF/Suspension/Double Wishbone Suspension ==
  Wheel : Inport
  Steering : Inport  Port=2
  Vehicle : Inport  Port=3
  Bus Creator1 : BusCreator  Inputs=5
  Bus Creator2 : BusCreator  Inputs=2
  Bus Creator3 : BusCreator  Inputs=2
  Bus Creator4 : BusCreator  Inputs=6
  Bus Selector : BusSelector  OutputSignals=z,Re,zdot,Fx,Fy,M
  Bus Selector1 : BusSelector  OutputSignals=P,V
  Independent Suspension – Double Wishbone : vehdynlibsuspension/Independent Suspension - Double Wishbone  ActiveDampEn=off  NumAxl=2  NumWhlsByAxl=[2 2]  StrgEnByAxl=[1 0]  AntiSwayEnByAxl=[1 0]  WhlNumVec="[1  2  1  2]"  AxleNumVec="[1  1  2  2]"  SuspTypesByAxle="[1  1]"  SuspImage=suspdw.png  IdealSuspEn=on  IdealSuspAxles="[1  2]"  Kz=Kz  F0z=F0z  Cz=Cz  Hmax=Hmax  f_act_susp_cz=[10000 10000;10000 10000]  f_act_susp_duty_bpt=[0 1]  f_act_susp_zdot_bpt=[-1 1]  Toe=0.  RollStrgSlp=0.  ToeStrgSlp=0.  Caster=0.  CasterHslp=0.  CasterStrgSlp=0.  Camber=0.  CamberHslp=0.  CamberStrgSlp=0.  StrgHgtSlp=0.1432  MappedSuspEn=off  MappedSuspAxles="[1  2]"  f_susp_axl_bp=[1 2]  f_susp_dz_bp=[-0.15 -0.14 -0.13 -0.12 -0.11 -0.10 -0.09 -0.08 -0.07 -0.06 -0.05 -0.04 -0.03 -0.02 -0.01 0.00 0.01 0.02 0.03 0.04 0.05 0.06 0.07 0.08 0.09 0.10 0.11 0.12 0.13 0.14 0.15]  f_susp_dzdot_bp=[-0.15 -0.14 -0.13 -0.12 -0.11 -0.10 -0.09 -0.08 -0.07 -0.06 -0.05 -0.04 -0.03 -0.02 -0.01 0.00 0.01 0.02 0.03 0.04 0.05 0.06 0.07 0.08 0.09 0.10 0.11 0.12 0.13 0.14 0.15]  f_susp_fmz=zeros(31,31,61,2,4)  f_susp_geom=zeros(31,61,2,3)  f_susp_strgdelta_bp=[-30,-29,-28,-27,-26,-25,-24,-23,-22,-21,-20,-19,-18,-17,-16,-15,-14,-13,-12,-11,-10,-9,-8,-7,-6,-5,-4,-3,-2,-1,0,1,2,3,4,5,6,7,8,9,10,11,12,13,14,15,16,17,18,19,20,21,22,23,24,25,26,27,28,29,30]  AntiSwayR=0.2  AntiSwayNtrlAng=0.5236  AntiSwayTrsK=8e2
  Selector1 : Selector  NumberOfDimensions=2  IndexOptions=Index vector (dialog),Select all  Indices=1,1  OutputSizes=1,1
  Selector2 : Selector  NumberOfDimensions=2  IndexOptions=Index vector (dialog),Select all  Indices=2,1  OutputSizes=1,1
  Steer Rate Adapter : Subsystem
  Steering Adapter : Subsystem
  Terminator : Terminator
  Vehicle Adapter : Subsystem
  Wheel  Adapter : Subsystem
  Suspension : Outport  VectorParamsAs1DForOutWhenUnconnected=off
  wires:
  Bus Selector/3 -> Independent Suspension – Double Wishbone/3  "<zdot>"
  Wheel  Adapter/1(WhlFx) -> Bus Creator4/1  "Fx"
  Bus Creator1/1 -> Bus Creator3/2  "Whl"
  Independent Suspension – Double Wishbone/6 -> Bus Creator1/4  "Ang"
  Wheel  Adapter/3(z) -> Bus Creator4/3
  Bus Selector/1 -> Independent Suspension – Double Wishbone/1  "<z>"
  Bus Selector/5 -> Independent Suspension – Double Wishbone/5  "<Fy>"
  Bus Selector/6 -> Independent Suspension – Double Wishbone/6  "<M>"
  Vehicle/1 -> Vehicle Adapter/1(Veh), Steer Rate Adapter/1(Veh)
  Wheel  Adapter/4(zdot) -> Bus Creator4/4
  Vehicle Adapter/1(VehSusp) -> Bus Selector1/1
  Independent Suspension – Double Wishbone/3 -> Bus Creator2/2  "M"
  Selector1/1 -> Bus Creator1/2  "xdot"
  Steering/1 -> Steering Adapter/1(Steer)
  Independent Suspension – Double Wishbone/4 -> Bus Creator1/1  "F"
  Bus Selector/4 -> Independent Suspension – Double Wishbone/4  "<Fx>"
  Wheel  Adapter/5(M) -> Bus Creator4/5  "M"
  Bus Selector/2 -> Independent Suspension – Double Wishbone/2  "<Re>"
  Independent Suspension – Double Wishbone/2 -> Bus Creator2/1  "F"
  Bus Selector1/2 -> Independent Suspension – Double Wishbone/8  "<V>"
  Selector2/1 -> Bus Creator1/3  "ydot"
  Independent Suspension – Double Wishbone/5 -> Selector1/1, Selector2/1  "V"
  Bus Creator2/1 -> Bus Creator3/1  "Veh"
  Bus Creator4/1 -> Bus Selector/1
  Steer Rate Adapter/1(AngVel) -> Bus Creator1/5  "AngVel"
  Wheel/1 -> Wheel  Adapter/1(Wheels)
  Wheel  Adapter/2(WhlFy) -> Bus Creator4/2  "Fy"
  Bus Selector1/1 -> Independent Suspension – Double Wishbone/7  "<P>"
  Wheel  Adapter/6(Re) -> Bus Creator4/6
  Independent Suspension – Double Wishbone/1 -> Terminator/1  "Susp"
  Steering Adapter/1(StrgAng) -> Independent Suspension – Double Wishbone/9
  Bus Creator3/1 -> Suspension/1

== system EV6_LUT_FourWheel_EV6Battery77p4kWh_PowerCorrected/Vehicle Under Test1/Vehicle/Vehicle Dynamics/Vehicle 14DOF/Suspension/Independent Mapped Front Suspension Mapped Solid Axle Rear Suspension ==
  Wheel : Inport
  Steering : Inport  Port=2
  Vehicle : Inport  Port=3
  Bus Creator1 : BusCreator  Inputs=5
  Bus Creator2 : BusCreator  Inputs=2
  Bus Creator3 : BusCreator  Inputs=2
  Bus Creator4 : BusCreator  Inputs=6
  Bus Selector : BusSelector  OutputSignals=z,Re,zdot,Fx,Fy,M
  Bus Selector1 : BusSelector  OutputSignals=P,V
  Independent Suspension - Mapped : vehdynlibsuspension/Independent Suspension - Mapped  NumAxl=1  NumWhlsByAxl=[2 2]  StrgEnByAxl=1  AntiSwayEnByAxl=1  WhlNumVec="[1  2  1  2]"  AxleNumVec="[1  1]"  SuspTypesByAxle=[2]  SuspImage=suspindmap.png  IdealSuspEn=off  IdealSuspAxles="[1  2]"  Kz=64370  F0z=9810  Cz=10000  Hmax=0.5  Toe=2  RollStrgSlp=-13  ToeStrgSlp=0.01  Caster=4  CasterHslp=-13  CasterStrgSlp=0.01  Camber=4  CamberHslp=-13  CamberStrgSlp=0.01  StrgHgtSlp=0.0025  MappedSuspEn=on  MappedSuspAxles=[1]  f_susp_axl_bp=[1 2]  f_susp_dz_bp=f_susp_dz_bp  f_susp_dzdot_bp=f_susp_dzdot_bp  f_susp_fmz=f_susp_fmz  f_susp_geom=f_susp_geom  f_susp_strgdelta_bp=f_susp_strgdelta_bp  NDFLookupOutType=1:4  NDGLookupOutType=1:3  AntiSwayR=0.2  AntiSwayNtrlAng=0.5236  AntiSwayTrsK=8e2
      link override For each track and axle combination calculate suspension forces and moments/Suspension/Suspension Angle Calculations: OverrideUsingVariant=MappedSteeringEnabled
      link override For each track and axle combination calculate suspension forces and moments/Suspension/Z axis suspension characteristic: OverrideUsingVariant=MappedSuspension
  Matrix Concatenate{,1..2,4..6} (6 alike) : Concatenate  Mode=Multidimensional array  ConcatenateDimension=2
  Selector1 : Selector  NumberOfDimensions=2  IndexOptions=Select all,Index vector (dialog)  Indices=[1 2],[3 4]  OutputSizes=1,1
  Selector10 : Selector  NumberOfDimensions=2  IndexOptions=Select all,Index vector (dialog)  Indices=[1 2],[1 2]  OutputSizes=1,1
  Selector11 : Selector  NumberOfDimensions=2  IndexOptions=Select all,Index vector (dialog)  Indices=[1 2],[1 2]  OutputSizes=1,1
  Selector12 : Selector  NumberOfDimensions=2  InputPortWidth=3  IndexOptions=Index vector (dialog),Select all  Indices=1,1  OutputSizes=1,1
  Selector13 : Selector  NumberOfDimensions=2  InputPortWidth=3  IndexOptions=Index vector (dialog),Select all  Indices=2,1  OutputSizes=1,1
  Selector14 : Selector  NumberOfDimensions=2  InputPortWidth=3  IndexOptions=Index vector (dialog),Select all  Indices=1,1  OutputSizes=1,1
  Selector15 : Selector  NumberOfDimensions=2  InputPortWidth=3  IndexOptions=Index vector (dialog),Select all  Indices=2,1  OutputSizes=1,1
  Selector{3,16,20..22} (5 alike) : Selector  IndexOptions=Index vector (dialog)  Indices=[3 4]  OutputSizes=1
  Selector17 : Selector  NumberOfDimensions=2  IndexOptions=Select all,Index vector (dialog)  Indices=[1 2],[3 4]  OutputSizes=1,1
  Selector18 : Selector  NumberOfDimensions=2  IndexOptions=Select all,Index vector (dialog)  Indices=[1 2],[3 4]  OutputSizes=1,1
  Selector{2,4..8} (6 alike) : Selector  IndexOptions=Index vector (dialog)  Indices=[1 2]  OutputSizes=1
  Selector9 : Selector  NumberOfDimensions=2  IndexOptions=Select all,Index vector (dialog)  Indices=[1 2],[1 2]  OutputSizes=1,1
  Solid Axle Suspension - Mapped : vehdynlibsuspension/Solid Axle Suspension - Mapped  NumAxl=1  NumWhlsByAxl=[2 2]  StrgEnByAxl=0  WhlNumVec="[1  2  1  2]"  AxleNumVec="[1  1]"  SuspTypesByAxle=[2]  SuspImage=suspsamap.png  AxlIxx=AxlIxx  AxlM=AxlM  TrackCoords=[0 0;VEH.TrackWidth*[-1 1]/2;0 0]  SuspCoords=[0 0;VEH.TrackWidth*[-1 1]/2;0 0]  KzWhlAxl=KzWhlAxl  F0zWhlAxl=F0zWhlAxl  CzWhlAxl=CzWhlAxl  IdealSuspEn=off  IdealSuspAxles="[1  2]"  Kz=64370  F0z=9810  Cz=10000  Hmax=0.5  Toe=2  RollStrgSlp=-13  ToeStrgSlp=0.01  Caster=4  CasterHslp=-13  CasterStrgSlp=0.01  Camber=4  CamberHslp=-13  CamberStrgSlp=0.01  StrgHgtSlp=0.0025  MappedSuspEn=on  MappedSuspAxles=[1]  f_susp_axl_bp=[1 2]  f_susp_dz_bp=f_susp_dz_bp  f_susp_dzdot_bp=f_susp_dzdot_bp  f_susp_fmz=f_susp_fmz  f_susp_geom=f_susp_geom  f_susp_strgdelta_bp=f_susp_strgdelta_bp  NDFLookupOutType=1:4  NDGLookupOutType=1:3
      link override For each track and axle combination calculate suspension forces and moments/Suspension/Suspension Angle Calculations: OverrideUsingVariant=MappedSteeringEnabled
      link override For each track and axle combination calculate suspension forces and moments/Suspension/Z axis suspension characteristic: OverrideUsingVariant=MappedSuspension
  Steer Rate Adapter : Subsystem
  Steering Adapter : Subsystem
  Terminator : Terminator
  Terminator1 : Terminator
  Vehicle Adapter : Subsystem
  Wheel  Adapter : Subsystem
  Suspension : Outport  VectorParamsAs1DForOutWhenUnconnected=off
  wires:
  Steer Rate Adapter/1(AngVel) -> Bus Creator1/5
  Bus Selector/2 -> Selector4/1, Selector20/1  "<Re>"
  Bus Creator3/1 -> Suspension/1
  Bus Creator1/1 -> Bus Creator3/2  "Whl"
  Bus Selector/5 -> Selector16/1, Selector8/1  "<Fy>"
  Bus Selector/1 -> Selector5/1, Selector3/1  "<z>"
  Solid Axle Suspension - Mapped/6 -> Matrix Concatenate2/2
  Bus Selector1/1 -> Selector1/1, Selector10/1  "<P>"
  Matrix Concatenate6/1 -> Bus Creator2/1  "F"
  Wheel  Adapter/6(Re) -> Bus Creator4/6
  Selector11/1 -> Independent Suspension - Mapped/8
  Wheel  Adapter/1(WhlFx) -> Bus Creator4/1  "Fx"
  Bus Selector/6 -> Selector17/1, Selector9/1  "<M>"
  Selector6/1 -> Independent Suspension - Mapped/3
  Steering Adapter/1(StrgAng) -> Selector2/1
  Vehicle Adapter/1(VehSusp) -> Bus Selector1/1
  Bus Selector1/2 -> Selector18/1, Selector11/1  "<V>"
  Selector3/1 -> Solid Axle Suspension - Mapped/1
  Selector15/1 -> Matrix Concatenate/2
  Matrix Concatenate1/1 -> Bus Creator1/2  "xdot"
  Steering/1 -> Steering Adapter/1(Steer)
  Matrix Concatenate/1 -> Bus Creator1/3  "ydot"
  Wheel  Adapter/5(M) -> Bus Creator4/5
  Selector2/1 -> Independent Suspension - Mapped/9
  Selector17/1 -> Solid Axle Suspension - Mapped/6
  Bus Creator4/1 -> Bus Selector/1
  Wheel  Adapter/2(WhlFy) -> Bus Creator4/2  "Fy"
  Matrix Concatenate2/1 -> Bus Creator1/4  "Ang"
  Independent Suspension - Mapped/5 -> Selector13/1, Selector12/1
  Bus Selector/4 -> Selector21/1, Selector7/1  "<Fx>"
  Bus Creator2/1 -> Bus Creator3/1  "Veh"
  Independent Suspension - Mapped/1 -> Terminator/1  "FSusp"
  Selector20/1 -> Solid Axle Suspension - Mapped/2
  Independent Suspension - Mapped/6 -> Matrix Concatenate2/1
  Independent Suspension - Mapped/2 -> Matrix Concatenate6/1
  Selector8/1 -> Independent Suspension - Mapped/5
  Independent Suspension - Mapped/3 -> Matrix Concatenate5/1
  Selector5/1 -> Independent Suspension - Mapped/1
  Wheel/1 -> Wheel  Adapter/1(Wheels)
  Solid Axle Suspension - Mapped/2 -> Matrix Concatenate6/2
  Wheel  Adapter/3(z) -> Bus Creator4/3
  Selector9/1 -> Independent Suspension - Mapped/6
  Selector10/1 -> Independent Suspension - Mapped/7
  Selector4/1 -> Independent Suspension - Mapped/2
  Independent Suspension - Mapped/4 -> Matrix Concatenate4/1
  Matrix Concatenate5/1 -> Bus Creator2/2  "M"
  Selector16/1 -> Solid Axle Suspension - Mapped/5
  Matrix Concatenate4/1 -> Bus Creator1/1  "F"
  Selector1/1 -> Solid Axle Suspension - Mapped/7
  Solid Axle Suspension - Mapped/3 -> Matrix Concatenate5/2
  Wheel  Adapter/4(zdot) -> Bus Creator4/4
  Vehicle/1 -> Vehicle Adapter/1(Veh), Steer Rate Adapter/1(Veh)
  Selector21/1 -> Solid Axle Suspension - Mapped/4
  Selector14/1 -> Matrix Concatenate1/2
  Selector13/1 -> Matrix Concatenate/1
  Selector18/1 -> Solid Axle Suspension - Mapped/8
  Selector7/1 -> Independent Suspension - Mapped/4
  Selector12/1 -> Matrix Concatenate1/1
  Solid Axle Suspension - Mapped/1 -> Terminator1/1  "Susp"
  Solid Axle Suspension - Mapped/4 -> Matrix Concatenate4/2
  Bus Selector/3 -> Selector6/1, Selector22/1  "<zdot>"
  Selector22/1 -> Solid Axle Suspension - Mapped/3
  Solid Axle Suspension - Mapped/5 -> Selector14/1, Selector15/1
